simulink model "SMTorqueControl_PdM"  (R2026a)
settings: Solver=FixedStepDiscrete  StopTime=1  FixedStep=Ts  EnableMultiTasking=on
PreLoadFcn:
  | if exist(fullfile(pwd, 'Ortak_Veri_ve_Parametreler'), 'dir'), addpath(fullfile(pwd, 'Ortak_Veri_ve_Parametreler')); end
  | if exist(fullfile(pwd, '..', 'Ortak_Veri_ve_Parametreler'), 'dir'), addpath(fullfile(pwd, '..', 'Ortak_Veri_ve_Parametreler')); end
  | if exist(fullfile(pwd, 'Mat_Dosyalari'), 'dir'), addpath(fullfile(pwd, 'Mat_Dosyalari')); end
  | SMTorqueControlData;
  | if ~exist('Cdc_PdM','var'), Cdc_PdM = Cdc; end;
  | if ~exist('ESR_PdM','var'), ESR_PdM = 1e-4; end;
  | if ~exist('Rbat_PdM','var'), Rbat_PdM = 1e-3; end;
  | if ~exist('Rs_PdM','var'), Rs_PdM = Rs; end;
  | if ~exist('Lad_PdM','var'), Lad_PdM = Lad; end;
  | if ~exist('Rfd_PdM','var'), Rfd_PdM = Rfd; end;
  | if ~exist('Gate_Fault_Mask','var'), Gate_Fault_Mask = [1;1;1;1;1;1]; end;
  | if ~exist('Stator_Unbalance_Gain','var'), Stator_Unbalance_Gain = [1;1;1]; end;
  | if ~exist('Load_Scale_PdM','var'), Load_Scale_PdM = 1.0; end;
  | if ~exist('Sensor_Offset_Drift_PdM','var'), Sensor_Offset_Drift_PdM = [0;0;0]; end;
InitFcn:
  | if exist(fullfile(pwd, 'Ortak_Veri_ve_Parametreler'), 'dir'), addpath(fullfile(pwd, 'Ortak_Veri_ve_Parametreler')); end
  | if exist(fullfile(pwd, '..', 'Ortak_Veri_ve_Parametreler'), 'dir'), addpath(fullfile(pwd, '..', 'Ortak_Veri_ve_Parametreler')); end
  | if exist(fullfile(pwd, 'Mat_Dosyalari'), 'dir'), addpath(fullfile(pwd, 'Mat_Dosyalari')); end
  | SMTorqueControlData;
  | if ~exist('Cdc_PdM','var'), Cdc_PdM = Cdc; end;
  | if ~exist('ESR_PdM','var'), ESR_PdM = 1e-4; end;
  | if ~exist('Rbat_PdM','var'), Rbat_PdM = 1e-3; end;
  | if ~exist('Rs_PdM','var'), Rs_PdM = Rs; end;
  | if ~exist('Lad_PdM','var'), Lad_PdM = Lad; end;
  | if ~exist('Rfd_PdM','var'), Rfd_PdM = Rfd; end;
  | if ~exist('Gate_Fault_Mask','var'), Gate_Fault_Mask = [1;1;1;1;1;1]; end;
  | if ~exist('Stator_Unbalance_Gain','var'), Stator_Unbalance_Gain = [1;1;1]; end;
  | if ~exist('Load_Scale_PdM','var'), Load_Scale_PdM = 1.0; end;
  | if ~exist('Sensor_Offset_Drift_PdM','var'), Sensor_Offset_Drift_PdM = [0;0;0]; end;
undefined symbols (not defined in the file): denZC_id, denZC_if, denZC_iq, ee_sli_rtmsupport, fsw, gcbh, Ibase, ID_MAP, IF_MAP, Ifbase, IQ_MAP, Kaw_id, Kaw_if, Kaw_iq, Ki_id, Ki_if, Ki_iq, Kp_id, Kp_if, Kp_iq, L_base, Lad, Ld, Lq, numZC_id, numZC_if, numZC_iq, p, Pmax, RPM_VECT, Tbase, TQ_VECT, Ts, Tsi, VDC_VECT, Vnom
libraries: nesl_utility x16, fl_lib x11, ee_lib x6, eeGeneralControl x3, eeTransforms x2, deeplib x2, sl_discontinuities x2, SignalEditorBlockLib x2, eeDqVoltageLimiter x1, simulink x1, sl_signal_attributes x1, eePwmGenerator x1
(part 2 of 2)

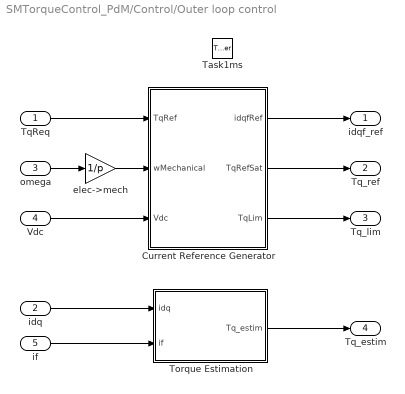
== system SMTorqueControl_PdM/Control/Outer loop control ==
  TqReq : Inport
  idq : Inport  Port=2
  omega : Inport  Port=3
  Vdc : Inport  Port=4
  if : Inport  Port=5
  Task1ms : TriggerPort  TriggerType=function-call  VariantControl=Variant  PortDimensions=1
  Current Reference Generator : Subsystem  LoadFcn=ee_sli_rtmsupport( 'loadfcn', gcbh );  mask(SM Current Reference Generator){Vnom=Vnom, Pmax=Pmax, Tmax=Tbase, ifmax=Ifbase, Ts=-1, RefType=Lookup-table based, rpmVec=RPM_VECT, TqVec=TQ_VECT, VdcVec=VDC_VECT, idMatrix=ID_MAP, iqMatrix=IQ_MAP, ifMatrix=IF_MAP, Kt=0.0375}
      mask prompts: Vnom "physmod:ee:library:comments:control:eeSmCurrentReferenceGen:NominalDclinkVoltageV_MP"; Pmax "physmod:ee:library:comments:control:eeSmCurrentReferenceGen:MaximumPowerW_MP"; Tmax "physmod:ee:library:comments:control:eeSmCurrentReferenceGen:MaximumTorqueNm_MP"; ifmax "physmod:ee:library:comments:control:eeSmCurrentReferenceGen:MaximumFieldCurrentA_MP"; Ts "physmod:ee:library:comments:control:eeSmCurrentReferenceGen:SampleTime1ForInherited_MP"; RefType "physmod:ee:library:comments:control:eeSmCurrentReferenceGen:CurrentReferences_MP"; rpmVec "physmod:ee:library:comments:control:eeSmCurrentReferenceGen:MechanicalSpeedVectorWMechanicalrpm_MP"; TqVec "physmod:ee:library:comments:control:eeSmCurrentReferenceGen:TorqueReferenceVectorTqRefNm_MP"; VdcVec "physmod:ee:library:comments:control:eeSmCurrentReferenceGen:DClinkVoltageVectorVdcV_MP"; idMatrix "physmod:ee:library:comments:control:eeSmCurrentReferenceGen:DaxisCurrentReferenceMatrixIdwMechanicalTqRefVdcA_MP"; iqMatrix "physmod:ee:library:comments:control:eeSmCurrentReferenceGen:QaxisCurrentReferenceMatrixIqwMechanicalTqRefVdcA_MP"; ifMatrix "physmod:ee:library:comments:control:eeSmCurrentReferenceGen:FieldCurrentReferenceMatrixIqwMechanicalTqRefVdcA_MP"; Kt "physmod:ee:library:comments:control:eeSmCurrentReferenceGen:TorqueConstantNmA_MP"
      mask help: physmod:ee:library:comments:control:eeSmCurrentReferenceGen:SMCurrentReferenceGenerator_MD
      mask init:
      | if Vnom <= 0            
      |     error(message('physmod:simscape:compiler:patterns:checks:GreaterThanZero',getString(message('physmod:ee:library:comments:control:eeSmCurrentReferenceGen:NominalDclinkVoltageV_MP'))));            
      | end
      | 
      | if Pmax <= 0            
      |     error(message('physmod:simscape:compiler:patterns:checks:GreaterThanZero',getString(message('physmod:ee:library:comments:control:eeSmCurrentReferenceGen:MaximumPowerW_MP'))));            
      | end
      | 
      | if Tmax <= 0            
      |     error(message('physmod:simscape:compiler:patterns:checks:GreaterThanZero',getString(message('physmod:ee:library:comments:control:eeSmCurrentReferenceGen:MaximumTorqueNm_MP'))));            
      | end
      | 
      | if ifmax <= 0            
      |     error(message('physmod:simscape:compiler:patterns:checks:GreaterThanZero',getString(message('physmod:ee:library:comments:control:eeSmCurrentReferenceGen:MaximumFieldCurrentA_MP'))));            
      | end
      | 
      | if RefType == 2
      | 	if length(rpmVec) < 2            
      | 		error(message('physmod:simscape:compiler:patterns:checks:LengthGreaterThanOrEqual',getString(message('physmod:ee:library:comments:control:eeSmCurrentReferenceGen:MechanicalSpeedVectorWMechanicalrpm_MP')), '2'));            
      |     end
      | 	if ~all(diff(rpmVec) > 0)            
      | 		error(message('physmod:simscape:compiler:patterns:checks:StrictlyAscendingVec',getString(message('physmod:ee:library:comments:control:eeSmCurrentReferenceGen:MechanicalSpeedVectorWMechanicalrpm_MP'))));            
      |     end
      |     if length(TqVec) < 2            
      |         error(message('physmod:simscape:compiler:patterns:checks:LengthGreaterThanOrEqual',getString(message('physmod:ee:library:comments:control:eeSmCurrentReferenceGen:TorqueReferenceVectorTqRefNm_MP')), '2'));            
      |     end
      |     if ~all(diff(TqVec) > 0)            
      |         error(message('physmod:simscape:compiler:patterns:checks:StrictlyAscendingVec',getString(message('physmod:ee:library:comments:control:eeSmCurrentReferenceGen:TorqueReferenceVectorTqRefNm_MP'))));            
      |     end
      | 	if length(VdcVec) < 2            
      |         error(message('physmod:simscape:compiler:patterns:checks:LengthGreaterThanOrEqual',getString(message('physmod:ee:library:comments:control:eeSmCurrentReferenceGen:DClinkVoltageVectorVdcV_MP')), '2'));            
      |     end
      | 	if ~all(diff(VdcVec) > 0)            
      |         error(message('physmod:simscape:compiler:patterns:checks:StrictlyAscendingVec',getString(message('physmod:ee:library:comments:control:eeSmCurrentReferenceGen:DClinkVoltageVectorVdcV_MP'))));            
      | 	end
      | 	if ~all(size(idMatrix) == [length(rpmVec), length(TqVec), length(VdcVec)])            
      |             error(message('physmod:simscape:compiler:patterns:checks:Size3DEqual',getString(message('physmod:ee:library:comments:control:eeSmCurrentReferenceGen:DaxisCurrentReferenceMatrixIdwMechanicalTqRefVdcA_MP')), getString(message('physmod:ee:library:comments:control:eeSmCurrentReferenceGen:MechanicalSpeedVectorWMechanicalrpm_MP')), getString(message('physmod:ee:library:comments:control:eeSmCurrentReferenceGen:TorqueReferenceVectorTqRefNm_MP')), getString(message('physmod:ee:library:comments:control:eeSmCurrentReferenceGen:DClinkVoltageVectorVdcV_MP'))));            
      |     end
      | 	if ~all(size(iqMatrix) == [length(rpmVec), length(TqVec), length(VdcVec)])            
      |         error(message('physmod:simscape:compiler:patterns:checks:Size3DEqual',getString(message('physmod:ee:library:comments:control:eeSmCurrentReferenceGen:QaxisCurrentReferenceMatrixIqwMechanicalTqRefVdcA_MP')), getString(message('physmod:ee:library:comments:control:eeSmCurrentReferenceGen:MechanicalSpeedVectorWMechanicalrpm_MP')), getString(message('physmod:ee:library:comments:control:eeSmCurrentReferenceGen:TorqueReferenceVectorTqRefNm_MP')), getString(message('physmod:ee:library:comments:control:eeSmCurrentReferenceGen:DClinkVoltageVectorVdcV_MP'))));            
      |     end
      | 	if ~all(size(ifMatrix) == [length(rpmVec), length(TqVec), length(VdcVec)])            
      |         error(message('physmod:simscape:compiler:patterns:checks:Size3DEqual',getString(message('physmod:ee:library:comments:control:eeSmCurrentReferenceGen:FieldCurrentReferenceMatrixIqwMechanicalTqRefVdcA_MP')), getString(message('physmod:ee:library:comments:control:eeSmCurrentReferenceGen:MechanicalSpeedVectorWMechanicalrpm_MP')), getString(message('physmod:ee:library:comments:control:eeSmCurrentReferenceGen:TorqueReferenceVectorTqRefNm_MP')), getString(message('physmod:ee:library:comments:control:eeSmCurrentReferenceGen:DClinkVoltageVectorVdcV_MP'))));            
      | 	end
      | end
      settings: CopyFcn=ee_sli_rtmsupport( 'copyfcn', gcbh );  DeleteFcn=ee_sli_rtmsupport( 'deletefcn', gcbh );  ModelCloseFcn=ee_sli_rtmsupport( 'modelclosefcn', gcbh );  PostSaveFcn=ee_sli_rtmsupport( 'postsavefcn', gcbh );  PreCopyFcn=ee_sli_rtmsupport( 'precopyfcn', gcbh );  OpenFcn=ee_sli_rtmsupport( 'openfcn', gcbh );  CloseFcn=ee_sli_rtmsupport( 'closefcn', gcbh );  PreDeleteFcn=ee_sli_rtmsupport( 'predeletefcn', gcbh );
      mask Help: web(nesl_help(gcbh))
      mask TypeOptions RefType: physmod:ee:library:comments:control:eeSmCurrentReferenceGen:ZeroD0x2DAxisControl_PV | physmod:ee:library:comments:control:eeSmCurrentReferenceGen:Lookup0x2DTableBased_PV
      mask Callback RefType: ee.mask.callbackPopupRefGenSm(gcb);
      mask DialogControl Container2 Prompt: physmod:ee:library:comments:control:eeSmCurrentReferenceGen:tab_GeneralParameters
      mask DialogControl Vnom Prompt: Nominal dc-link voltage (V)
      mask DialogControl Pmax Prompt: Maximum power (W)
      mask DialogControl Tmax Prompt: Maximum torque (N*m)
      mask DialogControl ifmax Prompt: Maximum field current (A)
      mask DialogControl Ts Prompt: Sample time (-1 for inherited)
      mask DialogControl Container3 Prompt: physmod:ee:library:comments:control:eeSmCurrentReferenceGen:tab_ReferenceGenStrategy
      mask DialogControl RefType Prompt: Current references
      mask DialogControl rpmVec Prompt: Mechanical speed vector, wMechanical (rpm)
      mask DialogControl TqVec Prompt: Torque reference vector, TqRef (N*m)
      mask DialogControl VdcVec Prompt: DC-link voltage vector, Vdc (V)
      mask DialogControl idMatrix Prompt: D-axis current reference matrix, id(wMechanical,TqRef,Vdc), (A)
      mask DialogControl iqMatrix Prompt: Q-axis current reference matrix, iq(wMechanical,TqRef,Vdc), (A)
      mask DialogControl ifMatrix Prompt: Field current reference matrix, iq(wMechanical,TqRef,Vdc), (A)
      mask DialogControl Kt Prompt: Torque constant (N*m/A)
  Torque Estimation : Subsystem
  elec->mech : Gain  Gain=1/p
  idqf_ref : Outport  VectorParamsAs1DForOutWhenUnconnected=off
  Tq_ref : Outport  Port=2  VectorParamsAs1DForOutWhenUnconnected=off
  Tq_lim : Outport  Port=3  VectorParamsAs1DForOutWhenUnconnected=off
  Tq_estim : Outport  Port=4  VectorParamsAs1DForOutWhenUnconnected=off
  wires:
  Torque Estimation/1(Tq_estim) -> Tq_estim/1
  idq/1 -> Torque Estimation/1(idq)
  if/1 -> Torque Estimation/2(if)
  Current Reference Generator/1(idqfRef) -> idqf_ref/1
  elec->mech/1 -> Current Reference Generator/2(wMechanical)
  Current Reference Generator/3(TqLim) -> Tq_lim/1
  Vdc/1 -> Current Reference Generator/3(Vdc)
  TqReq/1 -> Current Reference Generator/1(TqRef)
  omega/1 -> elec->mech/1
  Current Reference Generator/2(TqRefSat) -> Tq_ref/1

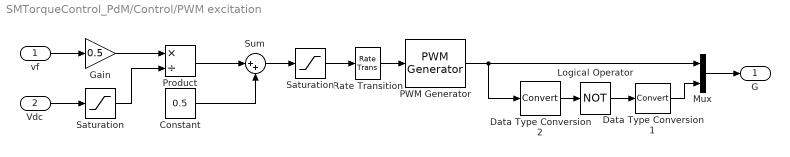
== system SMTorqueControl_PdM/Control/PWM excitation ==
  vf : Inport
  Vdc : Inport  Port=2
  Constant : Constant  Value=0.5  SampleTime=-1
  Data Type Conversion1 : DataTypeConversion  SaturateOnIntegerOverflow=off  RndMeth=Floor
  Data Type Conversion2 : DataTypeConversion  SaturateOnIntegerOverflow=off  RndMeth=Floor
  Gain : Gain  Gain=0.5
  Logical Operator : Logic  Operator=NOT  AllPortsSameDT=off  OutDataTypeStr=boolean
  Mux : Mux  Inputs=2
  PWM Generator : eePwmGenerator/PWM Generator  CarrCount=Up  Tper=1/fsw  Tdelay=0  Ts=Ts
  Product : Product  Inputs=*/
  Rate Transition : RateTransition
  Saturation : Saturate  UpperLimit=inf  LowerLimit=1
  "Saturation " : Saturate  UpperLimit=1  LowerLimit=0
  Sum : Sum  Inputs=|++
  G : Outport  VectorParamsAs1DForOutWhenUnconnected=off
  wires:
  vf/1 -> Gain/1
  Vdc/1 -> Saturation/1
  Saturation/1 -> Product/2
  Constant/1 -> Sum/2
  Sum/1 -> "Saturation "/1
  "Saturation "/1 -> Rate Transition/1
  Gain/1 -> Product/1
  Product/1 -> Sum/1
  Rate Transition/1 -> PWM Generator/1
  Data Type Conversion1/1 -> Mux/2
  PWM Generator/1 -> Data Type Conversion2/1, Mux/1
  Mux/1 -> G/1
  Data Type Conversion2/1 -> Logical Operator/1
  Logical Operator/1 -> Data Type Conversion1/1

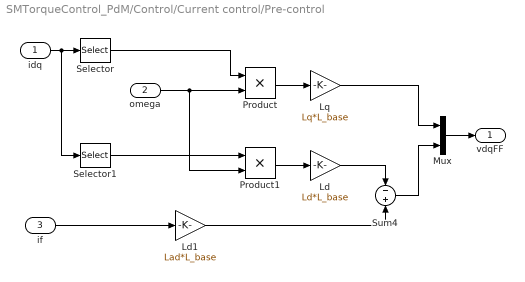
== system SMTorqueControl_PdM/Control/Current control/Pre-control ==
  idq : Inport
  omega : Inport  Port=2
  if : Inport  Port=3
  Ld : Gain  Gain=Ld*L_base
  Ld1 : Gain  Gain=Lad*L_base
  Lq : Gain  Gain=Lq*L_base
  Mux : Mux  Inputs=2
  Product : Product
  Product1 : Product
  Selector : Selector  InputPortWidth=2  IndexOptions=Index vector (dialog)  Indices=2  OutputSizes=1
  Selector1 : Selector  InputPortWidth=2  IndexOptions=Index vector (dialog)  Indices=1  OutputSizes=1
  Sum4 : Sum  Inputs=-+
  vdqFF : Outport  VectorParamsAs1DForOutWhenUnconnected=off
  wires:
  idq/1 -> Selector1/1, Selector/1
  Mux/1 -> vdqFF/1
  Selector1/1 -> Product1/1
  omega/1 -> Product1/2, Product/2
  Ld/1 -> Sum4/1
  if/1 -> Ld1/1
  Sum4/1 -> Mux/2
  Lq/1 -> Mux/1
  Ld1/1 -> Sum4/2
  Selector/1 -> Product/1
  Product1/1 -> Ld/1
  Product/1 -> Lq/1

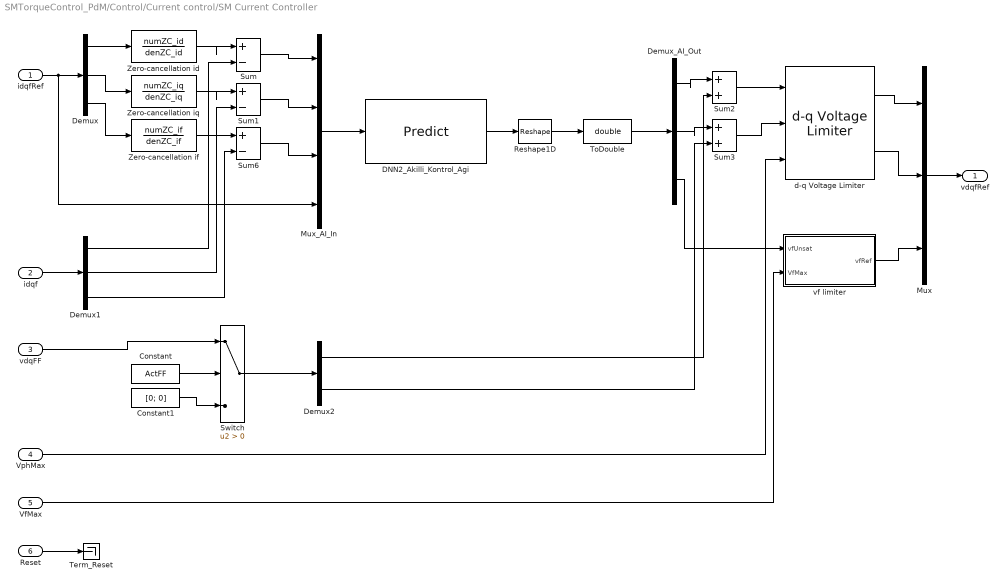
== system SMTorqueControl_PdM/Control/Current control/SM Current Controller ==
  idqfRef : Inport  SampleTime=Ts
  idqf : Inport  Port=2  SampleTime=Ts
  vdqFF : Inport  Port=3  SampleTime=Ts
  VphMax : Inport  Port=4  SampleTime=Ts
  VfMax : Inport  Port=5  SampleTime=Ts
  Reset : Inport  Port=6  SampleTime=Ts
  Constant : Constant  Value=ActFF  SampleTime=Ts
  Constant1 : Constant  Value=[0; 0]  SampleTime=Ts
  DNN2_Akilli_Kontrol_Agi : deeplib/Predict  Network=Network from MAT-file  NetworkFunction=squeezenet  NetworkFilePath=DNN2_ControllerNet.mat  MiniBatchSize=128  SimulateUsing=Interpreted execution  InputDataFormats={'Giris', 'CB';}  Predictions=on  Activations={}  ForceInterpretedSim=off  EnableDLNetwork=on  LastKnownNetworkFilePath='C:\Users\Dogukan.kilinc\OneDrive - figes.com.tr\Documents\MATLAB\Examples\R2026a\simscapeelectrical\SMTorqueControlExample\Mat_Dosyalari\DNN2_ControllerNet.mat'  LastKnownNetworkTimeStamp=740288.500960648176260292530059814453125
  Demux : Demux  Outputs=3
  Demux1 : Demux  Outputs=3
  Demux2 : Demux  Outputs=2
  Demux_AI_Out : Demux  Outputs=3
  Mux : Mux  Inputs=3
  Mux_AI_In : Mux
  Reshape1D : Reshape
  Sum : Sum  Inputs=|+-
  Sum1 : Sum  Inputs=|+-
  Sum2 : Sum  Inputs=|++
  Sum3 : Sum  Inputs=|++
  Sum6 : Sum  Inputs=|+-
  Switch : Switch  Criteria=u2 > Threshold  SaturateOnIntegerOverflow=off  InputSameDT=off  OutDataTypeStr=Inherit: Same as first input
  Term_Reset : Terminator
  ToDouble : DataTypeConversion  OutDataTypeStr=double  SaturateOnIntegerOverflow=off  RndMeth=Floor
  Zero-cancellation id : DiscreteTransferFcn  Numerator=numZC_id  Denominator=denZC_id  SampleTime=Ts
  Zero-cancellation if : DiscreteTransferFcn  Numerator=numZC_if  Denominator=denZC_if  SampleTime=Ts
  Zero-cancellation iq : DiscreteTransferFcn  Numerator=numZC_iq  Denominator=denZC_iq  SampleTime=Ts
  d-q Voltage Limiter : eeDqVoltageLimiter/d-q Voltage Limiter  AxisPrio=Q-axis  Ts=Ts
  vf limiter : Subsystem
  vdqfRef : Outport  VectorParamsAs1DForOutWhenUnconnected=off
  wires:
  idqfRef/1 -> Demux/1, Mux_AI_In/4
  idqf/1 -> Demux1/1
  Demux/1 -> Zero-cancellation id/1
  Demux/2 -> Zero-cancellation iq/1
  Demux/3 -> Zero-cancellation if/1
  Zero-cancellation id/1 -> Sum/1
  Zero-cancellation iq/1 -> Sum1/1
  Zero-cancellation if/1 -> Sum6/1
  Demux1/1 -> Sum/2
  Demux1/2 -> Sum1/2
  Demux1/3 -> Sum6/2
  Sum/1 -> Mux_AI_In/1
  Sum1/1 -> Mux_AI_In/2
  Sum6/1 -> Mux_AI_In/3
  Mux_AI_In/1 -> DNN2_Akilli_Kontrol_Agi/1
  DNN2_Akilli_Kontrol_Agi/1 -> Reshape1D/1
  Reshape1D/1 -> ToDouble/1
  ToDouble/1 -> Demux_AI_Out/1
  vdqFF/1 -> Switch/1
  Constant/1 -> Switch/2
  Constant1/1 -> Switch/3
  Switch/1 -> Demux2/1
  Demux_AI_Out/1 -> Sum2/1
  Demux_AI_Out/2 -> Sum3/1
  Demux2/1 -> Sum2/2
  Demux2/2 -> Sum3/2
  Sum2/1 -> d-q Voltage Limiter/1
  Sum3/1 -> d-q Voltage Limiter/2
  VphMax/1 -> d-q Voltage Limiter/3
  Demux_AI_Out/3 -> vf limiter/1(vfUnsat)
  VfMax/1 -> vf limiter/2(VfMax)
  d-q Voltage Limiter/1 -> Mux/1
  d-q Voltage Limiter/2 -> Mux/2
  vf limiter/1(vfRef) -> Mux/3
  Mux/1 -> vdqfRef/1
  Reset/1 -> Term_Reset/1

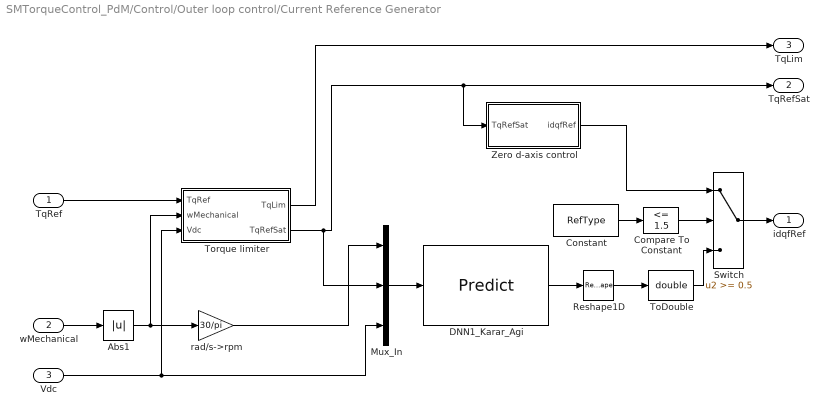
== system SMTorqueControl_PdM/Control/Outer loop control/Current Reference Generator ==
  TqRef : Inport  SampleTime=Ts
  wMechanical : Inport  Port=2  SampleTime=Ts
  Vdc : Inport  Port=3  SampleTime=Ts
  Abs1 : Abs  SaturateOnIntegerOverflow=off
  Compare To Constant : simulink/Logic and Bit Operations/Compare To Constant  relop=<=  const=1.5  OutDataTypeStr=boolean
  Constant : Constant  Value=RefType  SampleTime=Ts
  DNN1_Karar_Agi : deeplib/Predict  Network=Network from MAT-file  NetworkFunction=squeezenet  NetworkFilePath=DNN1_DecisionNet.mat  MiniBatchSize=128  SimulateUsing=Interpreted execution  InputDataFormats={'Giris', 'CB';}  Predictions=on  Activations={}  ForceInterpretedSim=off  EnableDLNetwork=on  LastKnownNetworkFilePath='C:\Users\Dogukan.kilinc\OneDrive - figes.com.tr\Documents\MATLAB\Examples\R2026a\simscapeelectrical\SMTorqueControlExample\Mat_Dosyalari\DNN1_DecisionNet.mat'  LastKnownNetworkTimeStamp=740288.500960648176260292530059814453125
  Mux_In : Mux  Inputs=3
  Reshape1D : Reshape
  Switch : Switch  Threshold=0.5  SaturateOnIntegerOverflow=off  InputSameDT=off
  ToDouble : DataTypeConversion  OutDataTypeStr=double  SaturateOnIntegerOverflow=off  RndMeth=Floor
  Torque limiter : Subsystem
  Zero d-axis control : Subsystem
  rad/s->rpm : Gain  Gain=30/pi
  idqfRef : Outport  VectorParamsAs1DForOutWhenUnconnected=off
  TqRefSat : Outport  Port=2  VectorParamsAs1DForOutWhenUnconnected=off
  TqLim : Outport  Port=3  VectorParamsAs1DForOutWhenUnconnected=off
  wires:
  Compare To Constant/1 -> Switch/2
  Zero d-axis control/1(idqfRef) -> Switch/1
  Torque limiter/2(TqRefSat) -> TqRefSat/1, Zero d-axis control/1(TqRefSat), Mux_In/2
  Torque limiter/1(TqLim) -> TqLim/1
  Abs1/1 -> Torque limiter/2(wMechanical), rad/s->rpm/1
  Switch/1 -> idqfRef/1
  TqRef/1 -> Torque limiter/1(TqRef)
  wMechanical/1 -> Abs1/1
  Vdc/1 -> Torque limiter/3(Vdc), Mux_In/3
  Constant/1 -> Compare To Constant/1
  rad/s->rpm/1 -> Mux_In/1
  Mux_In/1 -> DNN1_Karar_Agi/1
  DNN1_Karar_Agi/1 -> Reshape1D/1
  Reshape1D/1 -> ToDouble/1
  ToDouble/1 -> Switch/3

== system SMTorqueControl_PdM/Control/Outer loop control/Torque Estimation ==
  idq : Inport
  if : Inport  Port=2
  1/Ibase : Gain  Gain=1/Ibase
  1/Ifbase : Gain  Gain=1/Ifbase
  Demux : Demux  Outputs=2
  Gain : Gain  Gain=Lq-Ld
  Gain1 : Gain  Gain=Lad
  Product : Product
  Product1 : Product
  Sum : Sum  Inputs=|++
  Tbase : Gain  Gain=Tbase
  Tq_estim : Outport  VectorParamsAs1DForOutWhenUnconnected=off
  wires:
  idq/1 -> 1/Ibase/1
  Demux/1 -> Product/1
  Product/1 -> Gain/1
  Gain/1 -> Sum/1
  Demux/2 -> Product1/1, Product/2
  Product1/1 -> Gain1/1
  Sum/1 -> Tbase/1
  if/1 -> 1/Ifbase/1
  1/Ifbase/1 -> Product1/2
  1/Ibase/1 -> Demux/1
  Tbase/1 -> Tq_estim/1
  Gain1/1 -> Sum/2

== system SMTorqueControl_PdM/Control/Current control/SM Current Controller/vf limiter ==
  vfUnsat : Inport
  VfMax : Inport  Port=2
  Saturation Dynamic1 : sl_discontinuities/Saturation Dynamic  OutMin=[]  OutMax=[]  OutDataTypeStr=Inherit: Same as second input  OutDataType=fixdt(1, 16)  OutScaling=2^-10  DoSatur=off
  "Sign Change " : Gain  Gain=-1
  vfRef : Outport  VectorParamsAs1DForOutWhenUnconnected=off
  wires:
  Saturation Dynamic1/1 -> vfRef/1
  "Sign Change "/1 -> Saturation Dynamic1/3
  VfMax/1 -> "Sign Change "/1, Saturation Dynamic1/1
  vfUnsat/1 -> Saturation Dynamic1/2

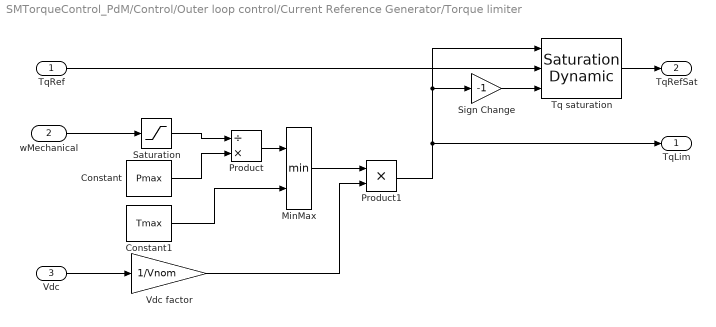
== system SMTorqueControl_PdM/Control/Outer loop control/Current Reference Generator/Torque limiter ==
  TqRef : Inport
  wMechanical : Inport  Port=2
  Vdc : Inport  Port=3
  Constant : Constant  Value=Pmax  SampleTime=Ts
  Constant1 : Constant  Value=Tmax  SampleTime=Ts
  MinMax : MinMax  Inputs=2  OutDataTypeStr=Inherit: Same as first input
  Product : Product  Inputs=/*  OutDataTypeStr=Inherit: Same as first input
  Product1 : Product
  Saturation : Saturate  UpperLimit=inf  LowerLimit=Pmax/Tmax
  Sign Change : Gain  Gain=-1
  Tq saturation : sl_discontinuities/Saturation Dynamic  OutMin=[]  OutMax=[]  OutDataTypeStr=Inherit: Same as second input  OutDataType=fixdt(1, 16)  OutScaling=2^-10  DoSatur=off
  Vdc factor : Gain  Gain=1/Vnom
  TqLim : Outport  VectorParamsAs1DForOutWhenUnconnected=off
  TqRefSat : Outport  Port=2  VectorParamsAs1DForOutWhenUnconnected=off
  wires:
  Constant/1 -> Product/2
  Saturation/1 -> Product/1
  Tq saturation/1 -> TqRefSat/1
  Product1/1 -> Tq saturation/1, Sign Change/1, TqLim/1
  TqRef/1 -> Tq saturation/2
  Vdc/1 -> Vdc factor/1
  Constant1/1 -> MinMax/2
  wMechanical/1 -> Saturation/1
  Product/1 -> MinMax/1
  Sign Change/1 -> Tq saturation/3
  MinMax/1 -> Product1/1
  Vdc factor/1 -> Product1/2

== system SMTorqueControl_PdM/Control/Outer loop control/Current Reference Generator/Zero d-axis control ==
  TqRefSat : Inport
  Abs : Abs  SaturateOnIntegerOverflow=off
  Data Type Conversion Inherited : sl_signal_attributes/Data Type Conversion Inherited  ConvertRealWorld=Real World Value  DoSatur=off
  Ifmin : Constant  Value=0.01*ifmax  SampleTime=Ts
  Kt : Gain  Gain=Kt
  MinMax : MinMax  Function=max  Inputs=2  OutDataTypeStr=Inherit: Same as first input
  Mux1 : Mux  Inputs=3
  Product : Product  Inputs=*/
  idRef : Constant  Value=0  SampleTime=Ts
  ifmax/Tmax : Gain  Gain=ifmax/Tmax
  idqfRef : Outport  VectorParamsAs1DForOutWhenUnconnected=off
  wires:
  idRef/1 -> Data Type Conversion Inherited/2
  Data Type Conversion Inherited/1 -> Mux1/1
  Ifmin/1 -> MinMax/2
  MinMax/1 -> Mux1/3, Kt/1
  Kt/1 -> Product/2
  ifmax/Tmax/1 -> MinMax/1
  Abs/1 -> ifmax/Tmax/1
  TqRefSat/1 -> Abs/1, Data Type Conversion Inherited/1, Product/1
  Product/1 -> Mux1/2
  Mux1/1 -> idqfRef/1

== stateflow chart SMTorqueControl_PdM/Control/Task scheduler ==
  (default) -> (junction 23) : CLK_50us
  (junction 23) -> (junction 17)
  (junction 17) -> (junction 22) [order 2]
  (junction 17) -> (junction 22) [order 1] : [cnt%%2==0]{Task_100us_1;}
  (junction 22) -> (junction 18) [order 2]
  (junction 22) -> (junction 18) [order 1] : [cnt%%2==0]{Task_100us_2;}
  (junction 18) -> (junction 21) [order 1] : [cnt%%20==0]{Task_1ms_1;}
  (junction 18) -> (junction 21) [order 2]
  (junction 21) -> (junction 34) [order 2]
  (junction 21) -> (junction 16) [order 1] : [1]{cnt++;}
  data: cnt local int32
  events: Task_100us_1 output FUNCTION_CALL_EVENT; Task_100us_2 output FUNCTION_CALL_EVENT; Task_1ms_1 output FUNCTION_CALL_EVENT; CLK_50us input FUNCTION_CALL_EVENT
